simulink model "Plant"  (R2018b)
settings: configuration reference "plant_config" (kept outside this file)
values from neighbouring files (symbols this model uses):
  PLANT_EXPORT = Simulink.Parameter(PLANT_EXPORT_VALUE)    [plant_model_init.m]
  PLANT_PARAM = Simulink.Parameter(PLANT_PARAM_VALUE)    [plant_model_init.m]
undefined symbols (not defined in the file or in its folder): acc_x, acc_x_O, acc_y, acc_y_O, acc_z, acc_z_O, alt, alt_0, day, DiscIntNeverNeededParam, fixType, flags, gSpeed, gyr_x, gyr_y, gyr_z, h_R, hAcc, heading, headingAcc, height, hMSL, hour, iTOW, lat, lon, M_BO, M_OB, mag_x, mag_y, mag_z, month, nano, numSV, pDOP, phi, PLANT_CONST, plant_model, pressure, prop_vel, psi, quat, reserved1, reserved2, rot_x_B, rot_y_B, rot_z_B, sAcc, sec, Sensor_Model, tAcc, temperature, temprature, theta, timestamp, vAcc, valid, vel_x_O, vel_y_O, vel_z_O ... (+6)
libraries: FMT_Model_Lib x13, dspsrcs4 x6, simulink x4, aerolibatmos2 x1
(part 2 of 2)

== system Plant/Sensor_Model/Sensor_MAG/Magnetometer/Physical_Model ==
  States : Inport
  Bus Selector : BusSelector  OutputSignals=Plant_States.lat,Plant_States.lon
  Bus Selector1 : BusSelector  OutputSignals=Extended_States.M_BO
  Product : Product  Multiplication=Matrix(*)  RndMeth=Zero  InputSameDT=on  OutDataTypeStr=Inherit: Same as first input
  WMM_LUT : Subsystem  mask{wmm_magnitude=Sensor_Model.Mag.WMM_Mag, wmm_declination=Sensor_Model.Mag.WMM_Dec, wmm_inclination=Sensor_Model.Mag.WMM_Inc, resolution=10}
      mask prompts: wmm_magnitude "WMM Magnitude Lookup Table"; wmm_declination "WMM Declination Lookup Table"; wmm_inclination "WMM Inclination Lookup Table"; resolution "Resolution (deg)"
  magnetic_field : Subsystem
  mag_B_gauss : Outport  Unit=T  PortDimensions=[3 1]
  wires:
  States/1 -> Bus Selector1/1, Bus Selector/1
  Bus Selector/2 -> WMM_LUT/2(lon_rad)  "<lon>"
  Bus Selector/1 -> WMM_LUT/1(lat_rad)  "<lat>"
  Bus Selector1/1 -> Product/1  "<M_BO>"
  Product/1 -> mag_B_gauss/1
  magnetic_field/1(mag_O_gauss) -> Product/2
  WMM_LUT/1(magnitude_uT) -> magnetic_field/1(magnitude_uT)
  WMM_LUT/2(declination_deg) -> magnetic_field/2(declination_deg)
  WMM_LUT/3(inclination_deg) -> magnetic_field/3(inclination_deg)

== system Plant/Sensor_Model/Sensor_MAG/Magnetometer/Sensor_Model ==
  Enable_Errors : Inport
  u : Inport  Port=2
  Add : Sum  InputSameDT=on  OutDataTypeStr=Inherit: Same as first input
  Saturation : Saturate  UpperLimit=Sensor_Model.Mag.Upper_limit  LowerLimit=Sensor_Model.Mag.Lower_limit
  Sensor_Error : Subsystem
  Sensor_Noise : Subsystem
  Switch : Switch  Criteria=u2 > Threshold
  y : Outport
  wires:
  Switch/1 -> y/1
  Saturation/1 -> Add/1
  Sensor_Error/1(y) -> Saturation/1
  Sensor_Noise/1(noise) -> Add/2
  Enable_Errors/1 -> Switch/2
  u/1 -> Switch/3, Sensor_Error/1(u)
  Add/1 -> Switch/1

== system Plant/Sensor_Model/Sensor_Barometer/Barometer/Sensor_Model/Sensor_Error ==
  u : Inport
  Constant3 : Constant  Value=Sensor_Model.Baro.Bias  VectorParams1D=off  OutDataTypeStr=single
  Sum : Sum  Inputs=|++  InputSameDT=on  OutDataTypeStr=Inherit: Same as first input
  y : Outport
  wires:
  Sum/1 -> y/1
  u/1 -> Sum/1
  Constant3/1 -> Sum/2

== system Plant/Sensor_Model/Sensor_Barometer/Barometer/Sensor_Model/Sensor_Noise ==
  Random Source : dspsrcs4/Random Source  SrcType=Gaussian  NormMethod=Ziggurat  CltLength=12  MinVal=0  MaxVal=1  MeanVal=0  VarVal=Sensor_Model.Baro.Variance  RepMode=Repeatable  rawSeed=1  IsInherit=off  SampMode=Discrete  SampTime=-1  SampFrame=1  DataType=Single  OutComplex=Real  OutputFrames=off
  noise : Outport
  wires:
  Random Source/1 -> noise/1

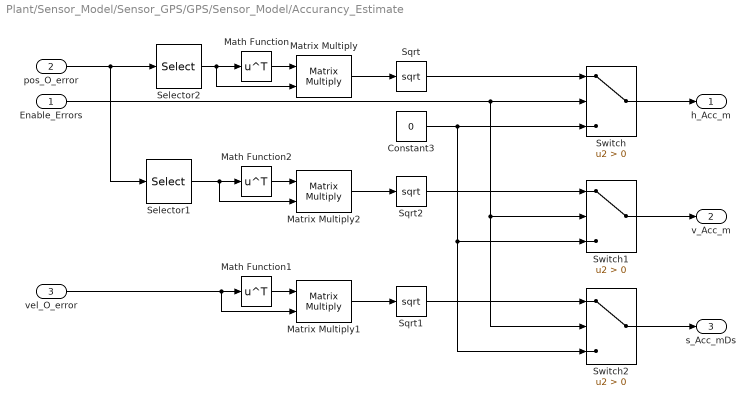
== system Plant/Sensor_Model/Sensor_GPS/GPS/Sensor_Model/Accurancy_Estimate ==
  Enable_Errors : Inport
  pos_O_error : Inport  Port=2
  vel_O_error : Inport  Port=3
  Constant3 : Constant  Value=0
  Math Function : Math  Operator=transpose  SaturateOnIntegerOverflow=on
  Math Function1 : Math  Operator=transpose  SaturateOnIntegerOverflow=on
  Math Function2 : Math  Operator=transpose  SaturateOnIntegerOverflow=on
  Matrix Multiply : Product  Multiplication=Matrix(*)
  Matrix Multiply1 : Product  Multiplication=Matrix(*)
  Matrix Multiply2 : Product  Multiplication=Matrix(*)
  Selector1 : Selector  InputPortWidth=3  IndexOptions=Index vector (dialog)  Indices=3  OutputSizes=1
  Selector2 : Selector  InputPortWidth=3  IndexOptions=Index vector (dialog)  Indices=[1 2]  OutputSizes=1
  Sqrt : Sqrt  OutputSignalType=real  SaturateOnIntegerOverflow=on
  Sqrt1 : Sqrt  OutputSignalType=real  SaturateOnIntegerOverflow=on
  Sqrt2 : Sqrt  OutputSignalType=real  SaturateOnIntegerOverflow=on
  Switch : Switch  Criteria=u2 > Threshold
  Switch1 : Switch  Criteria=u2 > Threshold
  Switch2 : Switch  Criteria=u2 > Threshold
  h_Acc_m : Outport
  v_Acc_m : Outport  Port=2
  s_Acc_mDs : Outport  Port=3
  wires:
  Switch/1 -> h_Acc_m/1
  pos_O_error/1 -> Selector1/1, Selector2/1
  Switch1/1 -> v_Acc_m/1
  Selector1/1 -> Math Function2/1, Matrix Multiply2/2
  Switch2/1 -> s_Acc_mDs/1
  Math Function1/1 -> Matrix Multiply1/1
  Math Function2/1 -> Matrix Multiply2/1
  Math Function/1 -> Matrix Multiply/1
  Selector2/1 -> Matrix Multiply/2, Math Function/1
  Matrix Multiply1/1 -> Sqrt1/1
  Matrix Multiply/1 -> Sqrt/1
  Matrix Multiply2/1 -> Sqrt2/1
  vel_O_error/1 -> Matrix Multiply1/2, Math Function1/1
  Sqrt/1 -> Switch/1
  Sqrt2/1 -> Switch1/1
  Enable_Errors/1 -> Switch2/2, Switch1/2, Switch/2
  Sqrt1/1 -> Switch2/1
  Constant3/1 -> Switch2/3, Switch1/3, Switch/3

== system Plant/Sensor_Model/Sensor_GPS/GPS/Sensor_Model/Sensor_Error ==
  Random Source : dspsrcs4/Random Source  SrcType=Gaussian  NormMethod=Ziggurat  CltLength=12  MinVal=0  MaxVal=1  MeanVal=0  VarVal=[0.2;0.2;0.4].^2  RepMode=Repeatable  rawSeed=1  IsInherit=off  SampMode=Discrete  SampTime=-1  SampFrame=1  DataType=Single  OutComplex=Real  OutputFrames=off
  Random Source1 : dspsrcs4/Random Source  SrcType=Gaussian  NormMethod=Ziggurat  CltLength=12  MinVal=0  MaxVal=1  MeanVal=0  VarVal=[0.01;0.01;0.01].^2  RepMode=Repeatable  rawSeed=1  IsInherit=off  SampMode=Discrete  SampTime=-1  SampFrame=1  DataType=Single  OutComplex=Real  OutputFrames=off
  pos_O_error : Outport
  vel_O_error : Outport  Port=2
  wires:
  Random Source/1 -> pos_O_error/1
  Random Source1/1 -> vel_O_error/1

== system Plant/Sensor_Model/Sensor_GPS/GPS/Sensor_Model/WGS84_Linearization ==
  WGS84_pos : Inport
  pos_O_error : Inport  Port=2
  Demux2 : Demux  Outputs=3
  Divide2 : Product  Inputs=/*
  LAT2FLAT Curve : FMT_Model_Lib/Transformation/LAT2FLAT Curve
      settings: SourceProductName=FMT Toolbox
  Terminator1 : Terminator
  Terminator2 : Terminator
  Vector Concatenate2 : Concatenate  NumInputs=3  Mode=Multidimensional array
  constant1 : Constant  Value=-1
  WGS84_pos_error : Outport
  wires:
  WGS84_pos/1 -> Demux2/1
  Demux2/1 -> LAT2FLAT Curve/1
  LAT2FLAT Curve/2 -> Vector Concatenate2/2
  pos_O_error/1 -> Divide2/2
  Vector Concatenate2/1 -> Divide2/1
  LAT2FLAT Curve/1 -> Vector Concatenate2/1
  Demux2/2 -> Terminator2/1
  Demux2/3 -> Terminator1/1
  constant1/1 -> Vector Concatenate2/3
  Divide2/1 -> WGS84_pos_error/1

== system Plant/Sensor_Model/Sensor_GPS/GPS/Sensor_Model/pos_filter ==
  pos_in : Inport
  Discrete FIR Filter : DiscreteFir
  pos_filter : Outport
  wires:
  Discrete FIR Filter/1 -> pos_filter/1
  pos_in/1 -> Discrete FIR Filter/1

== system Plant/Sensor_Model/Sensor_GPS/GPS/Sensor_Model/vel_filter ==
  vel_in : Inport
  Discrete FIR Filter : DiscreteFir
  vel_filter : Outport
  wires:
  Discrete FIR Filter/1 -> vel_filter/1
  vel_in/1 -> Discrete FIR Filter/1

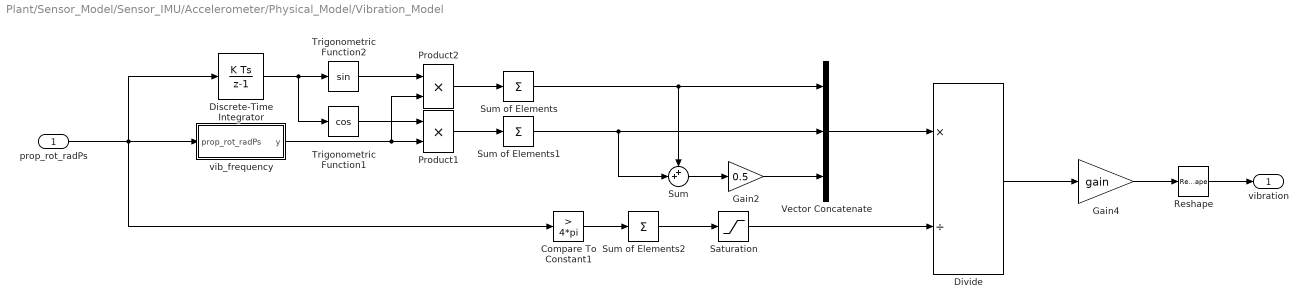
== system Plant/Sensor_Model/Sensor_IMU/Accelerometer/Physical_Model/Vibration_Model ==
  prop_rot_radPs : Inport  PortDimensions=[4,1]
  Compare To Constant1 : simulink/Logic and Bit Operations/Compare To Constant  relop=>  const=4*pi  OutDataTypeStr=boolean
  Discrete-Time Integrator : DiscreteIntegrator  InitialCondition=zeros(4,1)  SampleTime=-1  ICPrevOutput=DiscIntNeverNeededParam  ICPrevScaledInput=DiscIntNeverNeededParam
  Divide : Product  Inputs=*/
  Gain2 : Gain  Gain=0.5
  Gain4 : Gain  Gain=gain
  Product1 : Product  RndMeth=Zero
  Product2 : Product  RndMeth=Zero
  Reshape : Reshape  OutputDimensionality=Column vector (2-D)
  Saturation : Saturate  UpperLimit=8  LowerLimit=4
  Sum : Sum  Inputs=++|
  Sum of Elements : Sum  Inputs=+
  Sum of Elements1 : Sum  Inputs=+
  Sum of Elements2 : Sum  Inputs=+  CollapseMode=Specified dimension
  Trigonometric Function1 : Trigonometry  Operator=cos
  Trigonometric Function2 : Trigonometry
  Vector Concatenate : Concatenate  NumInputs=3  Mode=Multidimensional array
  vib_frequency : Subsystem
  vibration : Outport
  wires:
  Sum of Elements2/1 -> Saturation/1
  Saturation/1 -> Divide/2
  Divide/1 -> Gain4/1
  Compare To Constant1/1 -> Sum of Elements2/1
  Vector Concatenate/1 -> Divide/1
  Trigonometric Function1/1 -> Product1/1
  Trigonometric Function2/1 -> Product2/1
  Gain2/1 -> Vector Concatenate/3
  Sum/1 -> Gain2/1
  Sum of Elements1/1 -> Sum/2, Vector Concatenate/2
  Discrete-Time Integrator/1 -> Trigonometric Function1/1, Trigonometric Function2/1
  Sum of Elements/1 -> Vector Concatenate/1, Sum/1
  Reshape/1 -> vibration/1
  Gain4/1 -> Reshape/1
  prop_rot_radPs/1 -> Compare To Constant1/1, Discrete-Time Integrator/1, vib_frequency/1(prop_rot_radPs)
  vib_frequency/1(y) -> Product2/2, Product1/2
  Product2/1 -> Sum of Elements/1
  Product1/1 -> Sum of Elements1/1

== system Plant/Sensor_Model/Sensor_IMU/Accelerometer/Physical_Model/prop_vel ==
  States : Inport
  Bus Selector2 : BusSelector  OutputSignals=Extended_States.prop_vel
  Selector : Selector  InputPortWidth=8  IndexOptions=Index vector (dialog)  Indices=[1:4]  OutputSizes=1
  omega_radDs : Outport
  wires:
  States/1 -> Bus Selector2/1
  Bus Selector2/1 -> Selector/1  "<prop_vel>"
  Selector/1 -> omega_radDs/1

== system Plant/Sensor_Model/Sensor_IMU/Accelerometer/Physical_Model/specific_force ==
  States : Inport
  Bus Selector : BusSelector  OutputSignals=Plant_States.acc_x_O,Plant_States.acc_y_O,Plant_States.acc_z_O
  Bus Selector1 : BusSelector  OutputSignals=Extended_States.M_BO
  Gravity : Constant  Value=[0;0;Sensor_Model.g]  OutDataTypeStr=single
  Product1 : Product  Multiplication=Matrix(*)  RndMeth=Zero  InputSameDT=on  OutDataTypeStr=Inherit: Same as first input
  Sum : Sum  Inputs=|+-  InputSameDT=on  OutDataTypeStr=Inherit: Same as first input
  Vector Concatenate1 : Concatenate  NumInputs=3  Mode=Multidimensional array
  sfor_B_mPs2 : Outport  Unit=m/s^2
  wires:
  States/1 -> Bus Selector1/1, Bus Selector/1
  Bus Selector/1 -> Vector Concatenate1/1  "<acc_x_O>"
  Bus Selector/2 -> Vector Concatenate1/2  "<acc_y_O>"
  Bus Selector/3 -> Vector Concatenate1/3  "<acc_z_O>"
  Product1/1 -> sfor_B_mPs2/1
  Bus Selector1/1 -> Product1/1  "<M_BO>"
  Vector Concatenate1/1 -> Sum/1
  Sum/1 -> Product1/2
  Gravity/1 -> Sum/2

== system Plant/Sensor_Model/Sensor_IMU/Accelerometer/Sensor_Model/Sensor_Error ==
  u : Inport
  Add : Sum  InputSameDT=on  OutDataTypeStr=Inherit: Same as first input
  Constant : Constant  Value=eye(3)  OutDataTypeStr=single
  Constant1 : Constant  Value=Sensor_Model.Acc.Scalefactor_Error  VectorParams1D=off  OutDataTypeStr=single
  Constant3 : Constant  Value=Sensor_Model.Acc.Bias  VectorParams1D=off  OutDataTypeStr=single
  Product : Product  Multiplication=Matrix(*)  RndMeth=Zero  InputSameDT=on  OutDataTypeStr=Inherit: Same as first input
  Sum : Sum  Inputs=|++  InputSameDT=on  OutDataTypeStr=Inherit: Same as first input
  y : Outport
  wires:
  Sum/1 -> y/1
  Add/1 -> Product/1
  u/1 -> Product/2
  Constant1/1 -> Add/2
  Constant/1 -> Add/1
  Product/1 -> Sum/1
  Constant3/1 -> Sum/2

== system Plant/Sensor_Model/Sensor_IMU/Accelerometer/Sensor_Model/Sensor_Noise ==
  Random Source : dspsrcs4/Random Source  SrcType=Gaussian  NormMethod=Ziggurat  CltLength=12  MinVal=0  MaxVal=1  MeanVal=0  VarVal=Sensor_Model.Acc.Variance  RepMode=Repeatable  rawSeed=1  IsInherit=off  SampMode=Discrete  SampTime=-1  SampFrame=1  DataType=Single  OutComplex=Real  OutputFrames=off
  noise : Outport
  wires:
  Random Source/1 -> noise/1

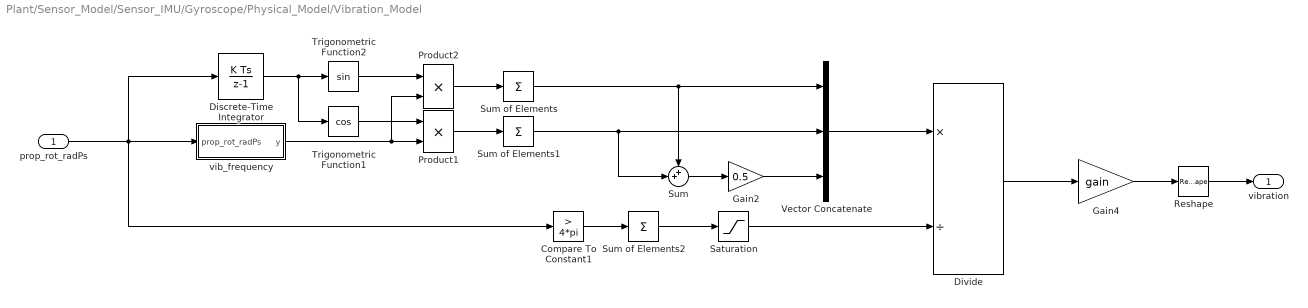
== system Plant/Sensor_Model/Sensor_IMU/Gyroscope/Physical_Model/Vibration_Model ==
  prop_rot_radPs : Inport  PortDimensions=[4,1]
  Compare To Constant1 : simulink/Logic and Bit Operations/Compare To Constant  relop=>  const=4*pi  OutDataTypeStr=boolean
  Discrete-Time Integrator : DiscreteIntegrator  InitialCondition=zeros(4,1)  SampleTime=-1  ICPrevOutput=DiscIntNeverNeededParam  ICPrevScaledInput=DiscIntNeverNeededParam
  Divide : Product  Inputs=*/
  Gain2 : Gain  Gain=0.5
  Gain4 : Gain  Gain=gain
  Product1 : Product  RndMeth=Zero
  Product2 : Product  RndMeth=Zero
  Reshape : Reshape  OutputDimensionality=Column vector (2-D)
  Saturation : Saturate  UpperLimit=8  LowerLimit=4
  Sum : Sum  Inputs=++|
  Sum of Elements : Sum  Inputs=+
  Sum of Elements1 : Sum  Inputs=+
  Sum of Elements2 : Sum  Inputs=+  CollapseMode=Specified dimension
  Trigonometric Function1 : Trigonometry  Operator=cos
  Trigonometric Function2 : Trigonometry
  Vector Concatenate : Concatenate  NumInputs=3  Mode=Multidimensional array
  vib_frequency : Subsystem
  vibration : Outport
  wires:
  Sum of Elements2/1 -> Saturation/1
  Saturation/1 -> Divide/2
  Divide/1 -> Gain4/1
  Compare To Constant1/1 -> Sum of Elements2/1
  Vector Concatenate/1 -> Divide/1
  Trigonometric Function1/1 -> Product1/1
  Trigonometric Function2/1 -> Product2/1
  Gain2/1 -> Vector Concatenate/3
  Sum/1 -> Gain2/1
  Sum of Elements1/1 -> Sum/2, Vector Concatenate/2
  Discrete-Time Integrator/1 -> Trigonometric Function1/1, Trigonometric Function2/1
  Sum of Elements/1 -> Vector Concatenate/1, Sum/1
  Reshape/1 -> vibration/1
  Gain4/1 -> Reshape/1
  prop_rot_radPs/1 -> Compare To Constant1/1, Discrete-Time Integrator/1, vib_frequency/1(prop_rot_radPs)
  vib_frequency/1(y) -> Product2/2, Product1/2
  Product2/1 -> Sum of Elements/1
  Product1/1 -> Sum of Elements1/1

== system Plant/Sensor_Model/Sensor_IMU/Gyroscope/Physical_Model/prop_vel ==
  States : Inport
  Bus Selector2 : BusSelector  OutputSignals=Extended_States.prop_vel
  Selector : Selector  InputPortWidth=8  IndexOptions=Index vector (dialog)  Indices=[1:4]  OutputSizes=1
  omega_radPs : Outport
  wires:
  Selector/1 -> omega_radPs/1
  States/1 -> Bus Selector2/1
  Bus Selector2/1 -> Selector/1  "<prop_vel>"

== system Plant/Sensor_Model/Sensor_IMU/Gyroscope/Physical_Model/rotation_speed ==
  States : Inport
  Bus Selector2 : BusSelector  OutputSignals=Plant_States.rot_x_B,Plant_States.rot_y_B,Plant_States.rot_z_B
  Vector Concatenate : Concatenate  NumInputs=3  Mode=Multidimensional array
  rot_radPs : Outport
  wires:
  Vector Concatenate/1 -> rot_radPs/1
  Bus Selector2/3 -> Vector Concatenate/3  "<rot_z_B>"
  Bus Selector2/1 -> Vector Concatenate/1  "<rot_x_B>"
  Bus Selector2/2 -> Vector Concatenate/2  "<rot_y_B>"
  States/1 -> Bus Selector2/1

== system Plant/Sensor_Model/Sensor_IMU/Gyroscope/Sensor_Model/Sensor_Error ==
  u : Inport
  Add : Sum  InputSameDT=on  OutDataTypeStr=Inherit: Same as first input
  Constant1 : Constant  Value=Sensor_Model.Gyro.Scalefactor_Error  VectorParams1D=off  OutDataTypeStr=single
  Constant2 : Constant  Value=eye(3)  OutDataTypeStr=single
  Constant3 : Constant  Value=Sensor_Model.Gyro.Bias  VectorParams1D=off  OutDataTypeStr=single
  Product : Product  Multiplication=Matrix(*)  RndMeth=Zero  InputSameDT=on  OutDataTypeStr=Inherit: Same as first input
  Sum : Sum  Inputs=|++  InputSameDT=on  OutDataTypeStr=Inherit: Same as first input
  y : Outport
  wires:
  Sum/1 -> y/1
  Product/1 -> Sum/1
  u/1 -> Product/2
  Add/1 -> Product/1
  Constant1/1 -> Add/2
  Constant2/1 -> Add/1
  Constant3/1 -> Sum/2

== system Plant/Sensor_Model/Sensor_IMU/Gyroscope/Sensor_Model/Sensor_Noise ==
  Random Source : dspsrcs4/Random Source  SrcType=Gaussian  NormMethod=Ziggurat  CltLength=12  MinVal=0  MaxVal=1  MeanVal=0  VarVal=Sensor_Model.Gyro.Variance  RepMode=Repeatable  rawSeed=1  IsInherit=off  SampMode=Discrete  SampTime=-1  SampFrame=1  DataType=Single  OutComplex=Real  OutputFrames=off
  noise : Outport
  wires:
  Random Source/1 -> noise/1

== system Plant/Sensor_Model/Sensor_MAG/Magnetometer/Physical_Model/WMM_LUT ==
  lat_rad : Inport
  lon_rad : Inport  Port=2
  Add : Sum
  Declination_Lookup_Table : LookupNDDirect  Table=wmm_declination  DiagnosticForOutOfRangeInput=Error
  Demux : Demux  Outputs=2
  Inclination_Lookup_Table : LookupNDDirect  Table=wmm_inclination  DiagnosticForOutOfRangeInput=Error
  Magnitude_Lookup_Table : LookupNDDirect  Table=wmm_magnitude  DiagnosticForOutOfRangeInput=Error
  Mux : Mux  Inputs=2
  Saturation1 : Saturate  UpperLimit=size(wmm_magnitude)-1  LowerLimit=0
  offset : Constant  Value=(size(wmm_magnitude)-1)/2  OutDataTypeStr=int32
  rad_to_index : Gain  Gain=180/pi/resolution  OutDataTypeStr=int32
  magnitude_uT : Outport
  declination_deg : Outport  Port=2
  inclination_deg : Outport  Port=3
  wires:
  Inclination_Lookup_Table/1 -> inclination_deg/1
  Declination_Lookup_Table/1 -> declination_deg/1
  Magnitude_Lookup_Table/1 -> magnitude_uT/1
  offset/1 -> Add/2
  Add/1 -> Saturation1/1
  rad_to_index/1 -> Add/1
  lat_rad/1 -> Mux/1
  lon_rad/1 -> Mux/2
  Mux/1 -> rad_to_index/1
  Saturation1/1 -> Demux/1
  Demux/1 -> Magnitude_Lookup_Table/1, Inclination_Lookup_Table/1, Declination_Lookup_Table/1
  Demux/2 -> Inclination_Lookup_Table/2, Magnitude_Lookup_Table/2, Declination_Lookup_Table/2

== system Plant/Sensor_Model/Sensor_MAG/Magnetometer/Physical_Model/magnetic_field ==
  magnitude_uT : Inport
  declination_deg : Inport  Port=2
  inclination_deg : Inport  Port=3
  Constant : Constant  Value=[1;0;0]  OutDataTypeStr=single
  Gain : Gain  Gain=-pi/180
  Gain1 : Gain  Gain=pi/180
  Multiply : Product
  Multiply1 : Product  Multiplication=Matrix(*)
  Multiply2 : Product  Multiplication=Matrix(*)
  Rotation Matrix Y : FMT_Model_Lib/Transformation/Rotation Matrix Y
      settings: SourceProductName=FMT Toolbox
  Rotation Matrix Z : FMT_Model_Lib/Transformation/Rotation Matrix Z
      settings: SourceProductName=FMT Toolbox
  toGauss : Gain  Gain=0.01
  mag_O_gauss : Outport
  wires:
  Constant/1 -> Multiply/2
  Multiply/1 -> Multiply1/2  "mag_field"
  Rotation Matrix Y/1 -> Multiply1/1
  inclination_deg/1 -> Gain/1
  Gain/1 -> Rotation Matrix Y/1
  declination_deg/1 -> Gain1/1
  Gain1/1 -> Rotation Matrix Z/1
  Rotation Matrix Z/1 -> Multiply2/1
  magnitude_uT/1 -> toGauss/1
  toGauss/1 -> Multiply/1  "magnitude_gauss"
  Multiply1/1 -> Multiply2/2
  Multiply2/1 -> mag_O_gauss/1

== system Plant/Sensor_Model/Sensor_MAG/Magnetometer/Sensor_Model/Sensor_Error ==
  u : Inport
  Add : Sum  InputSameDT=on  OutDataTypeStr=Inherit: Same as first input
  Constant : Constant  Value=eye(3)  OutDataTypeStr=single
  Constant1 : Constant  Value=Sensor_Model.Mag.Scalefactor_Error  VectorParams1D=off  OutDataTypeStr=single
  Constant3 : Constant  Value=Sensor_Model.Mag.Bias  VectorParams1D=off  OutDataTypeStr=single
  Product : Product  Multiplication=Matrix(*)  RndMeth=Zero  InputSameDT=on  OutDataTypeStr=Inherit: Same as first input
  Sum : Sum  Inputs=|++  InputSameDT=on  OutDataTypeStr=Inherit: Same as first input
  y : Outport
  wires:
  Sum/1 -> y/1
  Constant/1 -> Add/1
  Product/1 -> Sum/1
  u/1 -> Product/2
  Constant1/1 -> Add/2
  Add/1 -> Product/1
  Constant3/1 -> Sum/2

== system Plant/Sensor_Model/Sensor_MAG/Magnetometer/Sensor_Model/Sensor_Noise ==
  Random Source : dspsrcs4/Random Source  SrcType=Gaussian  NormMethod=Ziggurat  CltLength=12  MinVal=0  MaxVal=1  MeanVal=0  VarVal=Sensor_Model.Mag.Variance  RepMode=Repeatable  rawSeed=1  IsInherit=off  SampMode=Discrete  SampTime=-1  SampFrame=1  DataType=Single  OutComplex=Real  OutputFrames=off
  noise : Outport
  wires:
  Random Source/1 -> noise/1

== system Plant/Sensor_Model/Sensor_IMU/Accelerometer/Physical_Model/Vibration_Model/vib_frequency ==
  prop_rot_radPs : Inport
  Constant2 : Constant  Value=pi/30*1e4
  Divide2 : Product  Inputs=*/
  u^2 : Math  Operator=square  SaturateOnIntegerOverflow=on
  y : Outport
  wires:
  Divide2/1 -> u^2/1
  prop_rot_radPs/1 -> Divide2/1
  Constant2/1 -> Divide2/2
  u^2/1 -> y/1

== system Plant/Sensor_Model/Sensor_IMU/Gyroscope/Physical_Model/Vibration_Model/vib_frequency ==
  prop_rot_radPs : Inport
  Constant2 : Constant  Value=pi/30*1e4
  Divide2 : Product  Inputs=*/
  u^2 : Math  Operator=square  SaturateOnIntegerOverflow=on
  y : Outport
  wires:
  Divide2/1 -> u^2/1
  prop_rot_radPs/1 -> Divide2/1
  Constant2/1 -> Divide2/2
  u^2/1 -> y/1
